simulink model "rl_pi_tuner"  (R2026a)
settings: Solver=FixedStepDiscrete  StopTime=T_ep  FixedStep=Ts
model workspace (MATLAB code in the model file):
  | % Parameters (training randomises the virtual motor values in the reset function)
  | Ts = 0.01;              % controller / encoder sample time [s]
  | Ta = 3;                 % agent sample time = one reference step [s]
  | T_ep = 90;              % length of a training episode [s]
  | Vs = 12;                % controller output limit [V] (room for the x0.6 load, as on the hardware)
  | V_motor = 6;            % maximum voltage reaching the motor [V]
  | CPR = 12*298;           % encoder counts per output-shaft revolution
  | r_low = 70;  r_high = 90;  r_period = 6;   % speed reference [RPM], [s] (as on the hardware)
  | filt_num = 0.2;  filt_den = [1 -0.8];      % speed low-pass filter
  | logKp = [-2.5 0.3];     % Kp range, log10 (0.003 to 2 V/RPM)
  | logKi = [-1.3 0.9];     % Ki range, log10 (0.05 to 8 V/(RPM s))
  | 
  | % Virtual motor (nominal values; randomised during training)
  | K_true = 16;  tau_true = 0.054;  V_dead = 0.2;   % identified from the real motor (hw_id_noload2)
  | t_change = 40;  K_factor = 0.6;            % gain change part-way through
libraries: rllib x1
settings Model: Creator=00782620  LastModifiedBy=00782620

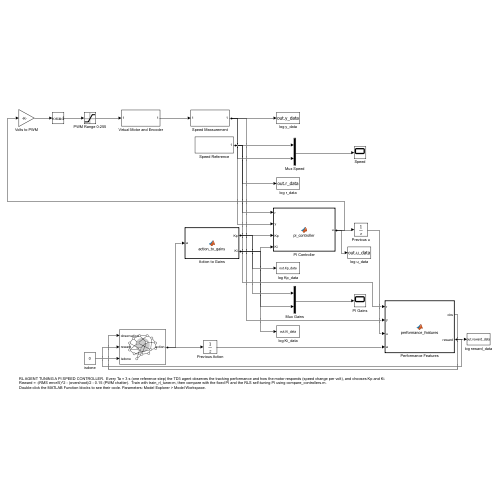
[thumbnail: Simulink's stored preview of the top-level diagram]
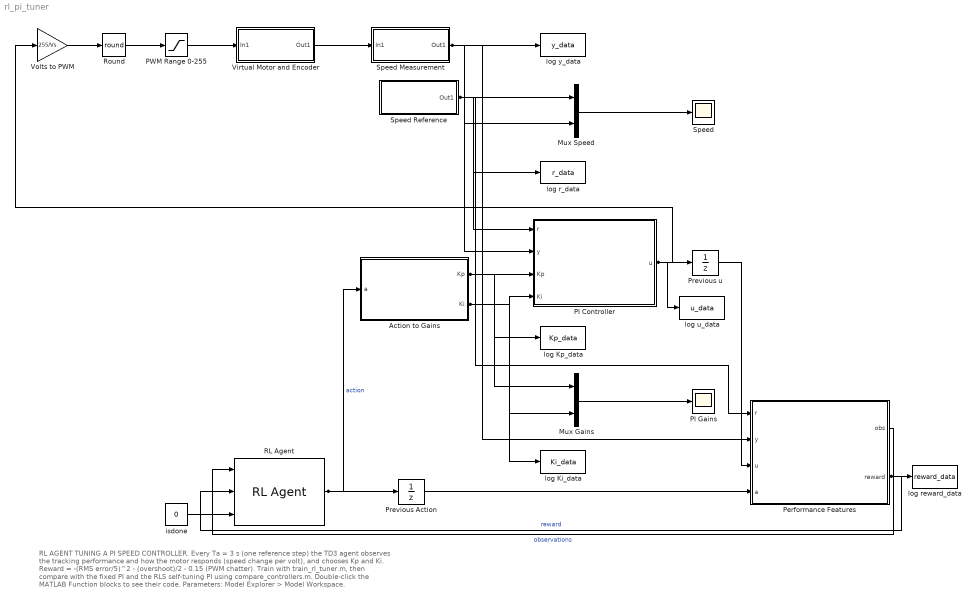
== system rl_pi_tuner ==
  note: RL AGENT TUNING A PI SPEED CONTROLLER.  Every Ta = 3 s (one reference step) the TD3 agent observes the tracking performance and how the motor responds (speed change per volt), and chooses Kp and Ki.
      | Reward = -(RMS error/5)^2 - (overshoot)/2 - 0.15 (PWM chatter).  Train with train_rl_tuner.m, then compare with the fixed PI and the RLS self-tuning PI using compare_controllers.m.
      | Double-click the MATLAB Function blocks to see their code. Parameters: Model Explorer > Model Workspace.
  Action to Gains : MATLAB Function  TreatAsAtomicUnit=on
  Mux Gains : Mux  Inputs=2
  Mux Speed : Mux  Inputs=2
  PI Controller : MATLAB Function  TreatAsAtomicUnit=on
  PI Gains : Scope
  PWM Range 0-255 : Saturate  UpperLimit=255  LowerLimit=0
  Performance Features : MATLAB Function  TreatAsAtomicUnit=on
  Previous Action : UnitDelay  InitialCondition=[0; 0]  SampleTime=Ts
  Previous u : UnitDelay  SampleTime=Ts
  RL Agent : rllib/RL Agent  Agent=agent  ExternalActionAsInput=off  ProvideLastAction=off  ProvideCumRwd=off  TreatAsDirectFeedthrough=on  UseStrictObservationDataTypes=off
  Round : Rounding  Operator=round
  Speed : Scope
  Speed Measurement : Subsystem
  Speed Reference : Subsystem
  Virtual Motor and Encoder : Subsystem
  Volts to PWM : Gain  Gain=255/Vs
  isdone : Constant  Value=0  SampleTime=Ta
  log Ki_data : ToWorkspace  VariableName=Ki_data  SampleTime=Ts
  log Kp_data : ToWorkspace  VariableName=Kp_data  SampleTime=Ts
  log r_data : ToWorkspace  VariableName=r_data  SampleTime=Ts
  log reward_data : ToWorkspace  VariableName=reward_data  SampleTime=Ts
  log u_data : ToWorkspace  VariableName=u_data  SampleTime=Ts
  log y_data : ToWorkspace  VariableName=y_data  SampleTime=Ts
  wires:
  Volts to PWM/1 -> Round/1
  Speed Reference/1(Out1) -> PI Controller/1(r), Mux Speed/1, Performance Features/1(r), log r_data/1
  Round/1 -> PWM Range 0-255/1
  Speed Measurement/1(Out1) -> PI Controller/2(y), Performance Features/2(y), Mux Speed/2, log y_data/1
  PWM Range 0-255/1 -> Virtual Motor and Encoder/1(In1)
  RL Agent/1 -> Previous Action/1, Action to Gains/1(a)  "action"
  isdone/1 -> RL Agent/3
  Virtual Motor and Encoder/1(Out1) -> Speed Measurement/1(In1)
  Action to Gains/1(Kp) -> Mux Gains/1, log Kp_data/1, PI Controller/3(Kp)
  Performance Features/1(obs) -> RL Agent/1  "observations"
  Mux Gains/1 -> PI Gains/1
  Action to Gains/2(Ki) -> PI Controller/4(Ki), Mux Gains/2, log Ki_data/1
  Previous Action/1 -> Performance Features/4(a)
  Mux Speed/1 -> Speed/1
  PI Controller/1(u) -> Previous u/1, Volts to PWM/1, log u_data/1
  Previous u/1 -> Performance Features/3(u)
  Performance Features/2(reward) -> RL Agent/2, log reward_data/1  "reward"

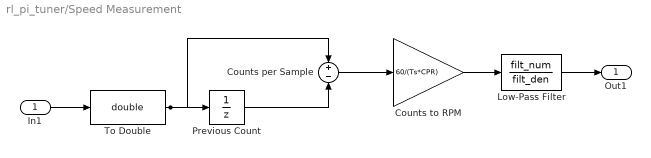
== system rl_pi_tuner/Speed Measurement ==
  In1 : Inport
  Counts per Sample : Sum  Inputs=+-
  Counts to RPM : Gain  Gain=60/(Ts*CPR)
  Low-Pass Filter : DiscreteFilter  Numerator=filt_num  Denominator=filt_den  SampleTime=Ts
  Previous Count : UnitDelay  SampleTime=Ts
  To Double : DataTypeConversion  OutDataTypeStr=double  SaturateOnIntegerOverflow=off  RndMeth=Floor
  Out1 : Outport
  wires:
  In1/1 -> To Double/1
  To Double/1 -> Previous Count/1, Counts per Sample/1
  Previous Count/1 -> Counts per Sample/2
  Counts per Sample/1 -> Counts to RPM/1
  Counts to RPM/1 -> Low-Pass Filter/1
  Low-Pass Filter/1 -> Out1/1

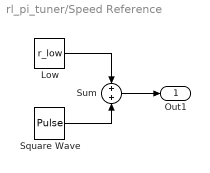
== system rl_pi_tuner/Speed Reference ==
  Low : Constant  Value=r_low  SampleTime=Ts
  Square Wave : DiscretePulseGenerator  Amplitude=r_high - r_low  Period=round(r_period/Ts)  PulseWidth=round(r_period/Ts/2)  PhaseDelay=round(r_period/Ts/2)  SampleTime=Ts
  Sum : Sum
  Out1 : Outport
  wires:
  Low/1 -> Sum/1
  Square Wave/1 -> Sum/2
  Sum/1 -> Out1/1

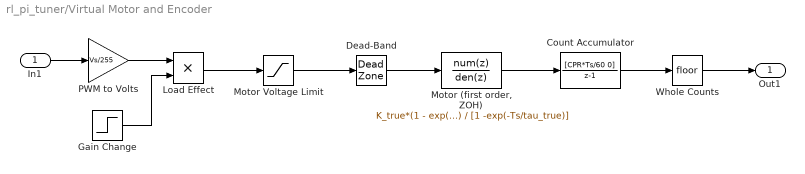
== system rl_pi_tuner/Virtual Motor and Encoder ==
  In1 : Inport
  Count Accumulator : DiscreteTransferFcn  Numerator=[CPR*Ts/60 0]  Denominator=[1 -1]  SampleTime=Ts
  Dead-Band : DeadZone  LowerValue=-V_dead  UpperValue=V_dead
  Gain Change : Step  Time=t_change  InitialValue=1  FinalValue=K_factor  SampleTime=Ts
  Load Effect : Product
  "Motor (first order, ZOH)" : DiscreteTransferFcn  Numerator=K_true*(1 - exp(-Ts/tau_true))  Denominator=[1 -exp(-Ts/tau_true)]  SampleTime=Ts
  Motor Voltage Limit : Saturate  UpperLimit=V_motor  LowerLimit=0
  PWM to Volts : Gain  Gain=Vs/255
  Whole Counts : Rounding
  Out1 : Outport
  wires:
  Count Accumulator/1 -> Whole Counts/1
  In1/1 -> PWM to Volts/1
  Motor Voltage Limit/1 -> Dead-Band/1
  Load Effect/1 -> Motor Voltage Limit/1
  Gain Change/1 -> Load Effect/2
  PWM to Volts/1 -> Load Effect/1
  Dead-Band/1 -> "Motor (first order, ZOH)"/1
  "Motor (first order, ZOH)"/1 -> Count Accumulator/1
  Whole Counts/1 -> Out1/1

== matlab function rl_pi_tuner/Performance Features ==
  data: r input; y input; u input; obs output; a input; reward output; Ts parameter; Ta parameter; Vs parameter
function [obs, reward] = performance_features(r, y, u, a, Ts, Ta, Vs)
% Observations and reward for the RL agent, over each agent interval Ta
% (one reference step).  At the end of each interval:
%
%   Khat = change in mean speed / change in mean voltage between this
%          interval and the last one.  This is how much the speed changes
%          per volt (an incremental gain, unaffected by the dead-band), so
%          it tells the agent when the motor has changed.
%   obs = [RMS error/10; overshoot/10; mean u/Vs; mean y/50; Khat/30;
%          previous Khat/30; previous RMS error/10; previous overshoot/10;
%          a(1); a(2)]
%   reward = -(RMS error/5)^2 - overshoot/2 - 0.15*chatter
%   chatter = mean |change in PWM duty| per sample (counts), which penalises
%   high gains that amplify encoder noise.
% where a is the agent's current action (the normalised PI gains).
% The values are held until the end of the next interval.
persistent n cnt sE2 osMax sU sY sDU uLast rLast dir obsH rewH Khat uMeanPrev yMeanPrev rmsPrev osPrev
if isempty(n)
    n = round(Ta/Ts);  cnt = 0;  sE2 = 0;  osMax = 0;  sU = 0;  sY = 0;  sDU = 0;  uLast = u;
    rLast = r;  dir = 0;  obsH = zeros(10, 1);  rewH = 0;
    Khat = 15;  uMeanPrev = 0;  yMeanPrev = 0;  rmsPrev = 0;  osPrev = 0;
end
y = double(y);
if cnt == 0                          % start of an interval: step direction
    dir = sign(r - rLast);
    rLast = r;
end
e = r - y;
sE2 = sE2 + e^2;
osMax = max(osMax, dir*(y - r));     % overshoot past the new reference
sU = sU + u;
sDU = sDU + abs(u - uLast);  uLast = u;
sY = sY + y;
cnt = cnt + 1;
if cnt >= n                          % end of the interval
    rmsE = sqrt(sE2/n);
    uMean = sU/n;  yMean = sY/n;
    KhatPrev = Khat;
    if abs(uMean - uMeanPrev) > 0.1   % incremental gain estimate
        Khat = min(max((yMean - yMeanPrev)/(uMean - uMeanPrev), 0), 90);
    end
    obsH = [rmsE/10; osMax/10; uMean/Vs; yMean/50; Khat/30; KhatPrev/30; ...
            rmsPrev/10; osPrev/10; a(1); a(2)];
    chatter = sDU/n*255/Vs;          % mean |change in PWM duty| [counts]
    rewH = -(rmsE/5)^2 - osMax/2 - 0.15*chatter;
    uMeanPrev = uMean;  yMeanPrev = yMean;  rmsPrev = rmsE;  osPrev = osMax;
    cnt = 0;  sE2 = 0;  osMax = 0;  sU = 0;  sY = 0;  sDU = 0;
end
obs = obsH;
reward = rewH;
end

== matlab function rl_pi_tuner/PI Controller ==
  data: r input; u output; y input; Kp input; Ki input; Ts parameter; Vs parameter
function u = pi_controller(r, y, Kp, Ki, Ts, Vs)
% Velocity-form PI controller with anti-windup (clamping)
%   u(k) = u(k-1) + (Kp + Ki*Ts)*e(k) - Kp*e(k-1),   0 <= u <= Vs
% The velocity form changes smoothly when the gains change.
persistent uPrev ePrev
if isempty(uPrev)
    uPrev = 0;  ePrev = 0;
end
e = r - double(y);
u = uPrev + (Kp + Ki*Ts)*e - Kp*ePrev;
u = min(max(u, 0), Vs);
uPrev = u;
ePrev = e;
end

== matlab function rl_pi_tuner/Action to Gains ==
  data: a input; Kp output; Ki output; logKp parameter; logKi parameter
function [Kp, Ki] = action_to_gains(a, logKp, logKi)
% Map the agent's action a in [-1, 1] to the PI gains, on a log scale
a = min(max(double(a), -1), 1);
Kp = 10^(logKp(1) + (a(1) + 1)/2*(logKp(2) - logKp(1)));
Ki = 10^(logKi(1) + (a(2) + 1)/2*(logKi(2) - logKi(1)));
end
